simulink model "CruiseControl"  (R2026b)
settings: Solver=ode4  StopTime=60
undefined symbols (not defined in the file): MphToMps
settings Model: DataDictionary=CruiseControlData.sldd  Creator=kingc  LastModifiedBy=kingc

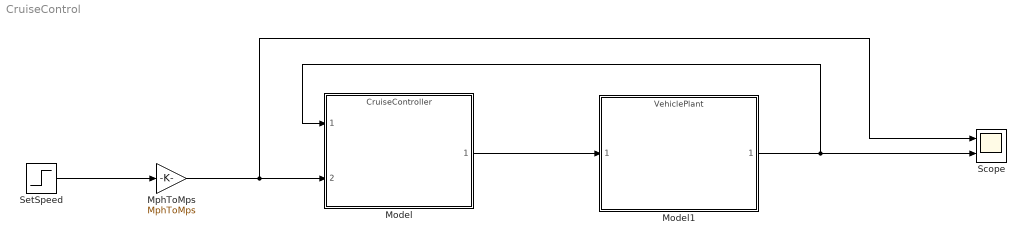
== system CruiseControl ==
  Model : ModelReference  ModelNameDialog=CruiseController.slx  SimulationMode=Normal  ModelReferenceVersion=1.3
  Model1 : ModelReference  ModelNameDialog=VehiclePlant.slx  SimulationMode=Normal  ModelReferenceVersion=1.5
  MphToMps : Gain  Gain=MphToMps
  Scope : Scope  NumInputPorts=2
  SetSpeed : Step  Time=5  FinalValue=65  SampleTime=0
  wires:
  SetSpeed/1 -> MphToMps/1
  MphToMps/1 -> Scope/1, Model/2
  Model/1 -> Model1/1
  Model1/1 -> Model/1, Scope/2
